simulink model "unit_recognize"  (R2026b)
settings: Solver=FixedStepDiscrete  EnableMultiTasking=on
values from neighbouring files (symbols this model uses):
  CONF_THRES = 0.5    [sign_detector.sldd]
  EDGE_PAD = 8.0    [sign_detector.sldd]
settings Model: DataDictionary=sign_detector.sldd  Creator=don  LastModifiedBy=don
settings SolverCC: PositivePriorityOrder=on
settings OptimizationCC: DifferentSizesBufferReuse=on  EfficientFloat2IntCast=on  EfficientTunableParamExpr=on  EnhancedBackFolding=on  LifeSpan=Inf  MaxStackSize=200000  OptimizationCustomize=off  OptimizeBlockOrder=speed  PassReuseOutputArgsAs=Individual arguments  UseDivisionForNetSlopeComputation=on
settings DebuggingCC: AlgebraicLoopMsg=error  ArtificialAlgebraicLoopMsg=error  AssertControl=DisableAll  BlockPriorityViolationMsg=error  BusObjectLabelMismatch=error  CheckMatrixSingularityMsg=error  InheritedTsInSrcMsg=error  IntegerOverflowMsg=error  IntegerSaturationMsg=error  ModelReferenceDataLoggingMessage=error  ModelReferenceIOMismatchMessage=error  NonBusSignalsTreatedAsBus=error  ParameterPrecisionLossMsg=error  ParameterTunabilityLossMsg=error  ParameterUnderflowMsg=error  ReadBeforeWriteMsg=EnableAllAsError  RootOutportRequireBusObject=error  SFcnCompatibilityMsg=error  SaveWithDisabledLinksMsg=error  SaveWithParameterizedLinksMsg=error  SigSpecEnsureSampleTimeMsg=error  SignalInfNanChecking=error  SignalLabelMismatchMsg=error  SignalRangeChecking=error  SolverPrmCheckMsg=error  StateNameClashWarn=warning  StrictBusMsg=ErrorOnBusTreatedAsVector  TasksWithSamePriorityMsg=error  UnconnectedInputMsg=error  UnconnectedLineMsg=error  UnconnectedOutputMsg=error  UnderSpecifiedDataTypeMsg=error  UniqueDataStoreMsg=error  UnknownTsInhSupMsg=error  UnnecessaryDatatypeConvMsg=warning  VariantConditionMismatch=error  VectorMatrixConversionMsg=error  WriteAfterReadMsg=EnableAllAsError  WriteAfterWriteMsg=EnableAllAsError
settings HardwareCC: ProdHWDeviceType=ARM Compatible->ARM Cortex-A (64-bit)  ProdLargestAtomicFloat=Double  ProdLargestAtomicInteger=LongLong  ProdLongLongMode=on
settings ModelReferenceCC: ModelReferenceNumInstancesAllowed=Single
settings SFSimCC: EnableRuntimeRecursion=off  MATLABDynamicMemAlloc=off  SimCustomHeaderCode="#include \"ncnn_infer.h\""  SimUserSources=ncnn_infer.cpp
settings SFSimCC: SimUserIncludeDirs=|
  | ../pi/ncnn
  | ../cache/ncnn_win/ncnn-20261020-windows-vs2026/x64/include
settings SFSimCC: SimUserLibraries=|
  | ../cache/ncnn_win/ncnn-20261020-windows-vs2026/x64/lib/ncnn.lib
  | ../cache/ncnn_win/ncnn-20261020-windows-vs2026/x64/lib/glslang.lib
  | ../cache/ncnn_win/ncnn-20261020-windows-vs2026/x64/lib/SPIRV.lib
  | ../cache/ncnn_win/ncnn-20261020-windows-vs2026/x64/lib/MachineIndependent.lib
  | ../cache/ncnn_win/ncnn-20261020-windows-vs2026/x64/lib/OSDependent.lib
  | ../cache/ncnn_win/ncnn-20261020-windows-vs2026/x64/lib/GenericCodeGen.lib
  | ../cache/ncnn_win/ncnn-20261020-windows-vs2026/x64/lib/glslang-default-resource-limits.lib
settings RTWCC: BuildConfiguration=Faster Runs  Description=Embedded Coder  HardwareBoard=Raspberry Pi (64bit)  PostCodeGenCommand=codertarget.postCodeGenHookCommand(h); pi_postcodegen(buildInfo)  SystemTargetFile=ert.tlc  TLCOptions="-aInlineSetEventsForThisBaseRateFcn=TLC_FALSE -aSuppressMultiTaskScheduler=TLC_FALSE  -aRateBasedStepFcn=0"  TargetLang=C++  TemplateMakefile=ert_default_tmf  Toolchain=GNU GCC RPIUtils
settings CodeAppCC: ForceParamTrailComments=on  IgnoreCustomStorageClasses=off  InsertBlockDesc=on  MATLABFcnDesc=on  MATLABSourceComments=on  OperatorAnnotations=on  ReqsInCode=on  SFDataObjDesc=on  SimulinkDataObjDesc=on  StateflowObjectComments=on
settings ERTTargetCC: CastingMode=Standards  CombineSignalStateStructs=on  EnableSignedLeftShifts=off  EnableSignedRightShifts=off  ExtModeIntrfLevel=Level2 - Open  ExtModeMexFile=ext_xcp  ExtModeStaticAlloc=on  GenerateSharedConstants=off  ParenthesesLevel=Standards  PreserveExpressionOrder=on  SubcomponentCodeInterfacePackaging=Nonreusable function  SupportNonFinite=off  SupportVariableSizeSignals=on  SuppressErrorStatus=on  TargetLangStandard=C++11 (ISO)  UtilityFuncGeneration=Shared location

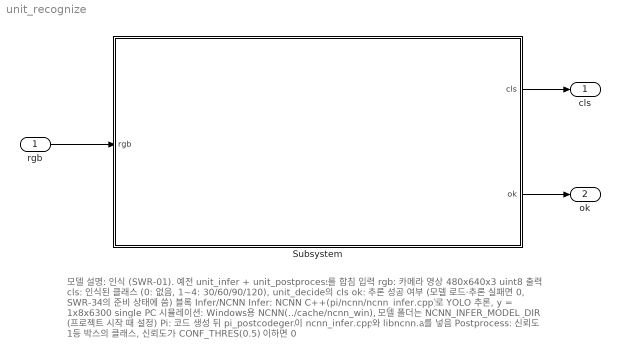
== system unit_recognize ==
  note: 모델 설명: 인식 (SWR-01). 예전 unit_infer + unit_postprocess를 합침
      | 입력
      | 	rgb: 카메라 영상 480x640x3 uint8
      | 출력
      | 	cls: 인식된 클래스 (0: 없음, 1~4: 30/60/90/120), unit_decide의 cls
      | 	ok: 추론 성공 여부 (모델 로드·추론 실패면 0, SWR-34의 준비 상태에 씀)
      | 블록
      | 	Infer/NCNN Infer: NCNN C++(pi/ncnn/ncnn_infer.cpp)로 YOLO 추론, y = 1x8x6300 single
      | 	  PC 시뮬레이션: Windows용 NCNN(../cache/ncnn_win), 모델 폴더는 NCNN_INFER_MODEL_DIR (프로젝트 시작 때 설정)
      | 	  Pi: 코드 생성 뒤 pi_postcodegen이 ncnn_infer.cpp와 libncnn.a를 넣음
      | 	Postprocess: 신뢰도 1등 박스의 클래스, 신뢰도가 CONF_THRES(0.5) 이하면 0
  rgb : Inport  OutDataTypeStr=uint8  PortDimensions=[480 640 3]  Interpolate=off
  Subsystem : Subsystem
  cls : Outport
  ok : Outport  Port=2
  wires:
  rgb/1 -> Subsystem/1(rgb)
  Subsystem/1(cls) -> cls/1
  Subsystem/2(ok) -> ok/1

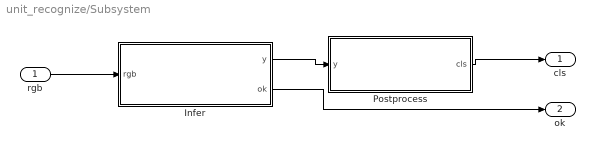
== system unit_recognize/Subsystem ==
  rgb : Inport
  Infer : Subsystem  Description=YOLO26n 추론 (NCNN C++, pi/ncnn/ncnn_infer.cpp). Pi와 PC 시뮬레이션이 같은 코드를 씀  VariantControl=(codegen)
  Postprocess : MATLAB Function  TreatAsAtomicUnit=on
  cls : Outport
  ok : Outport  Port=2
  wires:
  Infer/2(ok) -> ok/1
  Infer/1(y) -> Postprocess/1(y)
  Postprocess/1(cls) -> cls/1
  rgb/1 -> Infer/1(rgb)

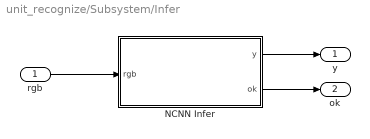
== system unit_recognize/Subsystem/Infer ==
  rgb : Inport
  NCNN Infer : MATLAB Function  TreatAsAtomicUnit=on
  y : Outport
  ok : Outport  Port=2
  wires:
  NCNN Infer/2(ok) -> ok/1
  NCNN Infer/1(y) -> y/1
  rgb/1 -> NCNN Infer/1(rgb)

== matlab function unit_recognize/Subsystem/Infer/NCNN Infer ==
  data: rgb input uint8; y output single; ok output boolean
function [y, ok] = infer_ncnn(rgb)

y = zeros(1, 8, 6300, 'single');
coder.cinclude('ncnn_infer.h');
status = int32(0);
status = coder.ceval('ncnn_infer', coder.rref(rgb), coder.wref(y));
ok = status == int32(0);
end

== matlab function unit_recognize/Subsystem/Postprocess ==
  data: y input; cls output double; CONF_THRES parameter double; EDGE_PAD parameter double
function cls = postprocess(y, CONF_THRES, EDGE_PAD)
%POSTPROCESS 추론 결과에서 표지판 1개를 고름 (SWR-01)
% 단위 모델 unit_recognize의 MATLAB Function 블록 "Postprocess" 코드
%   y:   1x8x6300 single (행 1~4: 박스 중심 x, 중심 y, 너비, 높이 [픽셀], 행 5~8: speed_30/60/90/120 점수)
%   cls: 신뢰도가 가장 높은 박스의 클래스 (1: speed_30, 2: speed_60, 3: speed_90, 4: speed_120)
%        그 신뢰도가 CONF_THRES 이하면 0 (표지판 없음)
%        그 박스가 화면 가장자리에서 EDGE_PAD 픽셀 안에 닿아도 0: 화면 밖으로 잘린 표지판은 테두리만 보여서
%        숫자를 잘못 읽기 쉽고, 표지판이 화면을 벗어나는 순간 틀린 값이 확정되면 다음 확정까지 남기 때문 (SWR-03)
%   한 프레임에서는 신뢰도가 가장 높은 표지판 1개만 씀 (SWR-01)
%#codegen
% 튜닝 상수 CONF_THRES, EDGE_PAD: 데이터 사전 models/sign_detector.sldd의 파라미터
IMG_W = 640;  % 모델 입력 너비 [픽셀] (pi/ncnn/ncnn_infer.cpp: 480x640)
IMG_H = 480;  % 모델 입력 높이 [픽셀]
p = reshape(y, 8, []);
[s, c] = max(p(5:8, :), [], 1);  % 박스마다 가장 높은 클래스 점수와 그 클래스
[conf, i] = max(s);              % 신뢰도 1등 박스
cls = 0;
if double(conf) > CONF_THRES
    b = double(p(1:4, i));       % 중심 x, 중심 y, 너비, 높이
    x0 = b(1) - b(3) / 2;
    x1 = b(1) + b(3) / 2;
    y0 = b(2) - b(4) / 2;
    y1 = b(2) + b(4) / 2;
    if x0 > EDGE_PAD && y0 > EDGE_PAD && x1 < IMG_W - EDGE_PAD && y1 < IMG_H - EDGE_PAD
        cls = double(c(i));      % MATLAB 인덱스가 1부터라 c가 이미 1~4
    end
end
end
